simulink model "b0_foc"  (R2023b)
settings: Solver=FixedStepDiscrete  StartTime=0.0  StopTime=150  FixedStep=0.001  RelTol=1e-3
undefined symbols (not defined in the file or in its folder): DiscIntNeverNeededParam
settings Model: Creator=28447  LastModifiedBy=28447
settings SFSimCC: SimCustomHeaderCode=extern void b0_ident_sim(float iq, float u, float omega, float e1, float v, float *b0, float *du);  SimUserIncludeDirs=D:\Desktop\RCESO\simulink
settings SFSimCC: SimUserSources=|
  | D:\Desktop\RCESO\simulink\b0_ident.c
  | D:\Desktop\RCESO\simulink\b0_ident_wrap.c

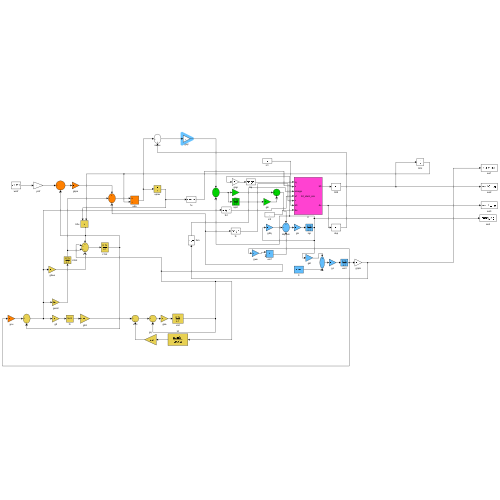
[thumbnail: Simulink's stored preview of the top-level diagram]
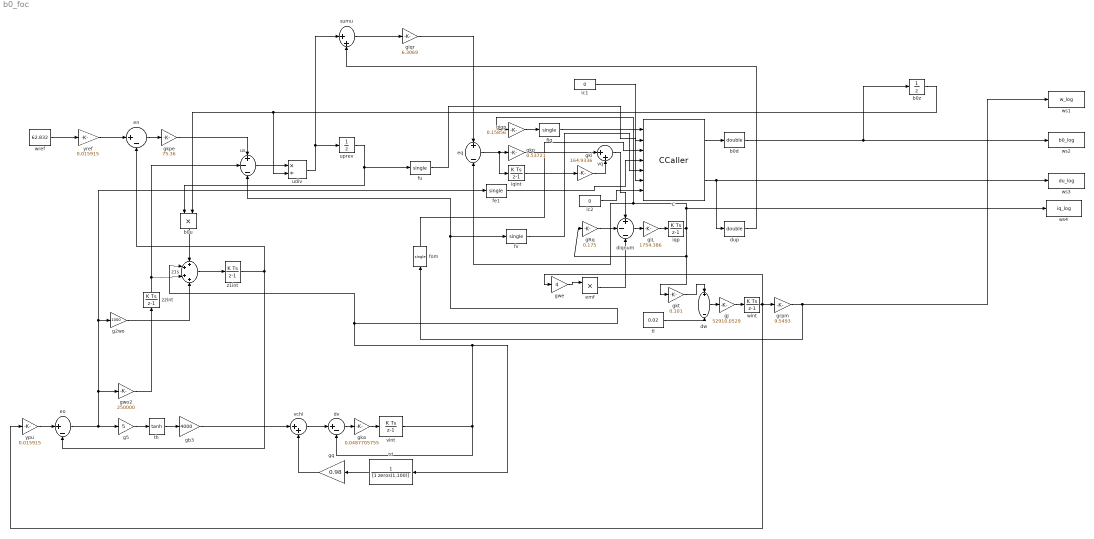
== system b0_foc ==
  C : CCaller  FunctionName=b0_ident_sim  PortSpecificationStruct="%)30     .    ^ L   8    (     @         %    \"     <    !     0         %  0 \"0    $    _    07)G3F%M90  4&]R=$YA;64 4V-O<&4     26YD97@     5'EP90      4VEZ90      27-';&]B86P   X    P    !@    @    $          4    (     0    (    !         !   @!I<0  #@   #     &    \"     0         !0    @    !     @    $         $  \" &EQ   .    .     8    (    !          %    \"     $    %     0         0  ...(+3754 chars)"
  b0d : DataTypeConversion  OutDataTypeStr=double  SaturateOnIntegerOverflow=off  RndMeth=Floor
  b0u : Product
  b0z : UnitDelay  InitialCondition=400  SampleTime=0.001  HasFrameUpgradeWarning=on
  diqnum : Sum  Inputs=+--
  dup : DataTypeConversion  OutDataTypeStr=double  SaturateOnIntegerOverflow=off  RndMeth=Floor
  dv : Sum  Inputs=|+-
  dw : Sum  Inputs=+-
  emf : Product
  en : Sum  Inputs=|+-
  eo : Sum  Inputs=|+-
  eq : Sum  Inputs=+-
  fe1 : DataTypeConversion  OutDataTypeStr=single  SaturateOnIntegerOverflow=off  RndMeth=Floor
  fiq : DataTypeConversion  OutDataTypeStr=single  SaturateOnIntegerOverflow=off  RndMeth=Floor
  fom : DataTypeConversion  OutDataTypeStr=single  SaturateOnIntegerOverflow=off  RndMeth=Floor
  fu : DataTypeConversion  OutDataTypeStr=single  SaturateOnIntegerOverflow=off  RndMeth=Floor
  fv : DataTypeConversion  OutDataTypeStr=single  SaturateOnIntegerOverflow=off  RndMeth=Floor
  g2wo : Gain  Gain=1000
  g5 : Gain  Gain=5
  gJ : Gain  Gain=52910.0529
  gRq : Gain  Gain=0.175
  gb3 : Gain  Gain=4000
  giL : Gain  Gain=1754.386
  giqp : Gain  Gain=0.15856
  giqr : Gain  Gain=6.3069
  gka : Gain  Gain=0.0487705755
  gki : Gain  Gain=164.9336
  gkp : Gain  Gain=0.53721
  gkpe : Gain  Gain=75.36
  gkt : Gain  Gain=0.101
  gq : Gain  Gain=0.98
  grpm : Gain  Gain=9.5493
  gwe : Gain  Gain=4
  gwo2 : Gain  Gain=250000
  ic1 : Constant  Value=0  OutDataTypeStr=single  SampleTime=0.001
  ic2 : Constant  Value=0  OutDataTypeStr=single  SampleTime=0.001
  iqint : DiscreteIntegrator  SampleTime=0.001  ICPrevOutput=DiscIntNeverNeededParam  ICPrevScaledInput=DiscIntNeverNeededParam
  iqp : DiscreteIntegrator  SampleTime=0.001  ICPrevOutput=DiscIntNeverNeededParam  ICPrevScaledInput=DiscIntNeverNeededParam
  sumu : Sum  Inputs=|++
  td : DiscreteTransferFcn  Numerator=1  Denominator=[1 zeros(1,100)]  SampleTime=0.001
  th : Trigonometry  Operator=tanh
  tl : Constant  Value=0.02  SampleTime=0.001
  udiv : Product  Inputs=*/
  uprev : UnitDelay  SampleTime=0.001  HasFrameUpgradeWarning=on
  us : Sum  Inputs=+--
  vchi : Sum  Inputs=|++
  vint : DiscreteIntegrator  SampleTime=0.001  ICPrevOutput=DiscIntNeverNeededParam  ICPrevScaledInput=DiscIntNeverNeededParam
  vq : Sum  Inputs=|++
  wint : DiscreteIntegrator  SampleTime=0.001  ICPrevOutput=DiscIntNeverNeededParam  ICPrevScaledInput=DiscIntNeverNeededParam
  wref : Constant  Value=62.832  SampleTime=0.001
  ws1 : ToWorkspace  VariableName=w_log  SaveFormat=Timeseries  SampleTime=0.001
  ws2 : ToWorkspace  VariableName=b0_log  SaveFormat=Timeseries  SampleTime=0.001
  ws3 : ToWorkspace  VariableName=du_log  SaveFormat=Timeseries  SampleTime=0.001
  ws4 : ToWorkspace  VariableName=iq_log  SaveFormat=Timeseries  SampleTime=0.001
  ypu : Gain  Gain=0.015915
  yref : Gain  Gain=0.015915
  z1int : DiscreteIntegrator  SampleTime=0.001  ICPrevOutput=DiscIntNeverNeededParam  ICPrevScaledInput=DiscIntNeverNeededParam
  z1s : Sum  Inputs=++++
  z2int : DiscreteIntegrator  SampleTime=0.001  ICPrevOutput=DiscIntNeverNeededParam  ICPrevScaledInput=DiscIntNeverNeededParam
  wires:
  giqp/1 -> fiq/1
  fiq/1 -> C/1
  uprev/1 -> b0u/1, fu/1
  fu/1 -> C/2
  grpm/1 -> ws1/1, fom/1
  fom/1 -> C/3
  eo/1 -> g5/1, fe1/1, g2wo/1, gwo2/1
  fe1/1 -> C/4
  vint/1 -> dv/2, fv/1, us/3, z1s/2, td/1
  fv/1 -> C/5
  ic1/1 -> C/6
  ic2/1 -> C/7
  C/1 -> b0d/1
  b0d/1 -> b0z/1, ws2/1
  C/2 -> dup/1, ws3/1
  udiv/1 -> sumu/1, uprev/1
  dup/1 -> sumu/2
  iqp/1 -> eq/2, giqp/1, ws4/1, gRq/1, gkt/1
  wref/1 -> yref/1
  yref/1 -> en/1
  z1int/1 -> en/2, eo/2
  en/1 -> gkpe/1
  gkpe/1 -> us/1
  z2int/1 -> us/2, z1s/3
  us/1 -> udiv/1
  b0z/1 -> udiv/2, b0u/2
  wint/1 -> gwe/1, ypu/1, grpm/1
  ypu/1 -> eo/1
  g5/1 -> th/1
  th/1 -> gb3/1
  td/1 -> gq/1
  gb3/1 -> vchi/1
  gq/1 -> vchi/2
  vchi/1 -> dv/1
  dv/1 -> gka/1
  gka/1 -> vint/1
  g2wo/1 -> z1s/4
  b0u/1 -> z1s/1
  z1s/1 -> z1int/1
  gwo2/1 -> z2int/1
  sumu/1 -> giqr/1
  giqr/1 -> eq/1
  eq/1 -> iqint/1, gkp/1
  iqint/1 -> gki/1
  gkp/1 -> vq/1
  gki/1 -> vq/2
  vq/1 -> diqnum/1
  gRq/1 -> diqnum/2
  emf/1 -> diqnum/3
  diqnum/1 -> giL/1
  giL/1 -> iqp/1
  gwe/1 -> emf/1
  gkt/1 -> dw/1
  tl/1 -> dw/2
  dw/1 -> gJ/1
  gJ/1 -> wint/1
